simulink model "VoltageSourceConverterHVDCTrans"  (R2025b)
settings: Solver=FixedStepDiscrete  StartTime=0.0  StopTime=5  FixedStep=Ts  MaxStep=1e-4  RelTol=1e-3
PreLoadFcn:
  | VoltageSourceConverterHVDCTransParameters
values from neighbouring files (symbols this model uses):
  c = 0.207e-6    (= 2.07e-07)    [VoltageSourceConverterHVDCTransParameters.m]
  Cf = ((QRatedFilter/(VRated^2*(2*pi*FRated)))*(n^2-1)/(n^2))/Cbase    [VoltageSourceConverterHVDCTransParameters.m]
  FRated = 60    [VoltageSourceConverterHVDCTransParameters.m]
  Idcbase = Pbase/VdcRated    (= 1000)    [VoltageSourceConverterHVDCTransParameters.m]
  IL0 = opIdc.get("I").Value.value    [VoltageSourceConverterHVDCTransInitializeModel.m]
  l = 0.189e-3    (= 0.000189)    [VoltageSourceConverterHVDCTransParameters.m]
  Lbase = Zbase/wbase    [VoltageSourceConverterHVDCTransParameters.m]
  Lr = 0.15    [VoltageSourceConverterHVDCTransParameters.m]
  n = 25    [VoltageSourceConverterHVDCTransParameters.m]
  PRated = 300e6    (= 300000000)    [VoltageSourceConverterHVDCTransParameters.m]
  r = 0.0376    [VoltageSourceConverterHVDCTransParameters.m]
  Rc = r*Dis    (= 11.28)    [VoltageSourceConverterHVDCTransParameters.m]
  Rr = 0.002    [VoltageSourceConverterHVDCTransParameters.m]
  Rt = 0.002625    [VoltageSourceConverterHVDCTransParameters.m]
  Ts = 1/(fsw*100)    [VoltageSourceConverterHVDCTransInitializeModel.m]    (also in VoltageSourceConverterHVDCTransParameters.m = 6.66666666667e-05; VoltageSourceConverterHVDCTransVariantControl.m)
  Tsc = 10*Ts    (= 0.166666666667)    [VoltageSourceConverterHVDCTransInitializeModel.m]    (also in VoltageSourceConverterHVDCTransParameters.m = 6.66666666667e-05; VoltageSourceConverterHVDCTransVariantControl.m)
  Vdcr0 = 2*opReceivingEndVdcp.get("V").Value.value    [VoltageSourceConverterHVDCTransInitializeModel.m]
  VdcRated = 300e3    (= 300000)    [VoltageSourceConverterHVDCTransParameters.m]
  Vdcs0 = 2*opSendingEndVdcp.get("V").Value.value    [VoltageSourceConverterHVDCTransInitializeModel.m]
  VRated = 150e3    (= 150000)    [VoltageSourceConverterHVDCTransParameters.m]
  Xt = 0.19197    [VoltageSourceConverterHVDCTransParameters.m]
  Zbase = Vbase/Ibase    [VoltageSourceConverterHVDCTransParameters.m]
undefined symbols (not defined in the file or in its folder): DiscIntNeverNeededParam
libraries: nesl_utility x43, fl_lib x32, ee_lib x22, eeTransforms x16, eeGeneralControl x14, slpidlib x13, mcbeeMathTransformLib x8, eeSinusoidalMeasurement x2, eePwmGeneratorThreeLevel x2
(part 3 of 4)

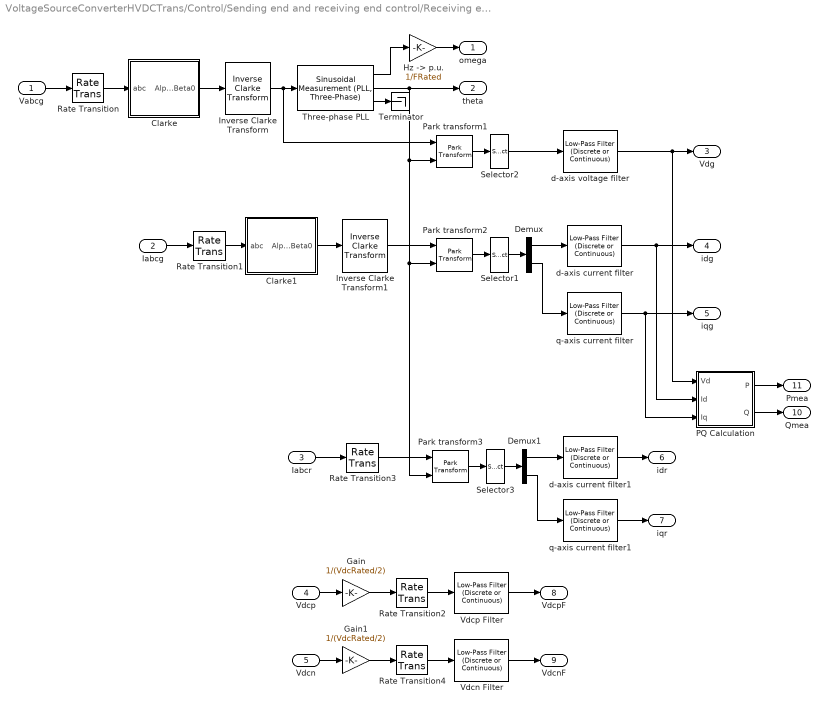
== system VoltageSourceConverterHVDCTrans/Control/Sending end and receiving end control/Receiving end control/Time mode/Measurements ==
  Vabcg : Inport
  Iabcg : Inport  Port=2
  Iabcr : Inport  Port=3
  Vdcp : Inport  Port=4
  Vdcn : Inport  Port=5
  Clarke : Subsystem
  Clarke1 : Subsystem
  Demux : Demux  Outputs=2
  Demux1 : Demux  Outputs=2
  Gain : Gain  Gain=1/(VdcRated/2)
  Gain1 : Gain  Gain=1/(VdcRated/2)
  "Hz -> p.u." : Gain  Gain=1/FRated
  Inverse Clarke Transform : mcbeeMathTransformLib/Inverse Clarke Transform  PowerInvariant=off  UseWithEmbedded=off  PhaseInput=Two inputs
      settings: LibrarySourceBlock=|
      | ee_sl_lib/Mathematical
      | Transforms/Inverse
      | Clarke Transform
  Inverse Clarke Transform1 : mcbeeMathTransformLib/Inverse Clarke Transform  PowerInvariant=off  UseWithEmbedded=off  PhaseInput=Two inputs
      settings: LibrarySourceBlock=|
      | ee_sl_lib/Mathematical
      | Transforms/Inverse
      | Clarke Transform
  PQ Calculation : Subsystem
  Park transform1 : eeTransforms/Park Transform  AxisAlignment=Q-axis  PowerInvariant=off
  Park transform2 : eeTransforms/Park Transform  AxisAlignment=Q-axis  PowerInvariant=off
  Park transform3 : eeTransforms/Park Transform  AxisAlignment=Q-axis  PowerInvariant=off
  Rate Transition : RateTransition  InitialCondition=Vabcgr0  OutPortSampleTime=Tsc
  Rate Transition1 : RateTransition  InitialCondition=Iabcgs0  OutPortSampleTime=Tsc
  Rate Transition2 : RateTransition  InitialCondition=Vdcr0/2/(VdcRated/2)  OutPortSampleTime=Tsc
  Rate Transition3 : RateTransition  InitialCondition=Iabcrs0  OutPortSampleTime=Tsc
  Rate Transition4 : RateTransition  InitialCondition=Vdcr0/2/(VdcRated/2)  OutPortSampleTime=Tsc
  Selector1 : Selector  InputPortWidth=3  IndexOptions=Index vector (dialog)  Indices=[1 2]  OutputSizes=1
  Selector2 : Selector  InputPortWidth=3  IndexOptions=Index vector (dialog)  Indices=[1]  OutputSizes=1
  Selector3 : Selector  InputPortWidth=3  IndexOptions=Index vector (dialog)  Indices=[1 2]  OutputSizes=1
  Terminator : Terminator
  Three-phase PLL : eeSinusoidalMeasurement/Sinusoidal Measurement (PLL, Three-Phase)  Kp_LF=45  Ki_LF=1250  F0=60  Theta0=-pi/6+Vphaser0  Ts=Tsc
  Vdcn Filter : eeGeneralControl/Low-Pass Filter (Discrete or Continuous)  K=1  T=5e-3  B=inf  A=-inf  init_option=Specify as parameter  x0=Vdcr0/2/(VdcRated/2)  Ts=Tsc
  Vdcp Filter : eeGeneralControl/Low-Pass Filter (Discrete or Continuous)  K=1  T=5e-3  B=inf  A=-inf  init_option=Specify as parameter  x0=Vdcr0/2/(VdcRated/2)  Ts=Tsc
  d-axis current filter : eeGeneralControl/Low-Pass Filter (Discrete or Continuous)  K=1  T=5e-3  B=inf  A=-inf  init_option=Specify as parameter  x0=Idgr0  Ts=Tsc
  d-axis current filter1 : eeGeneralControl/Low-Pass Filter (Discrete or Continuous)  K=1  T=5e-3  B=inf  A=-inf  init_option=Specify as parameter  x0=Idr0  Ts=Tsc
  d-axis voltage filter : eeGeneralControl/Low-Pass Filter (Discrete or Continuous)  K=1  T=5e-3  B=inf  A=-inf  init_option=Specify as parameter  x0=Vdgr0  Ts=Tsc
  q-axis current filter : eeGeneralControl/Low-Pass Filter (Discrete or Continuous)  K=1  T=5e-3  B=inf  A=-inf  init_option=Specify as parameter  x0=Iqgr0  Ts=Tsc
  q-axis current filter1 : eeGeneralControl/Low-Pass Filter (Discrete or Continuous)  K=1  T=5e-3  B=inf  A=-inf  init_option=Specify as parameter  x0=Iqr0  Ts=Tsc
  omega : Outport  VectorParamsAs1DForOutWhenUnconnected=off
  theta : Outport  Port=2  VectorParamsAs1DForOutWhenUnconnected=off
  Vdg : Outport  Port=3  VectorParamsAs1DForOutWhenUnconnected=off
  idg : Outport  Port=4  VectorParamsAs1DForOutWhenUnconnected=off
  iqg : Outport  Port=5  VectorParamsAs1DForOutWhenUnconnected=off
  idr : Outport  Port=6  VectorParamsAs1DForOutWhenUnconnected=off
  iqr : Outport  Port=7  VectorParamsAs1DForOutWhenUnconnected=off
  VdcpF : Outport  Port=8  VectorParamsAs1DForOutWhenUnconnected=off
  VdcnF : Outport  Port=9  VectorParamsAs1DForOutWhenUnconnected=off
  Qmea : Outport  Port=10  VectorParamsAs1DForOutWhenUnconnected=off
  Pmea : Outport  Port=11  VectorParamsAs1DForOutWhenUnconnected=off
  wires:
  Vdcn Filter/1 -> VdcnF/1
  Vdcn/1 -> Gain1/1
  Rate Transition4/1 -> Vdcn Filter/1
  Gain1/1 -> Rate Transition4/1
  q-axis current filter1/1 -> iqr/1
  d-axis current filter1/1 -> idr/1
  Demux1/2 -> q-axis current filter1/1
  Demux1/1 -> d-axis current filter1/1
  Rate Transition3/1 -> Park transform3/1
  Selector3/1 -> Demux1/1
  Park transform3/1 -> Selector3/1
  Iabcr/1 -> Rate Transition3/1
  PQ Calculation/2(Q) -> Qmea/1
  PQ Calculation/1(P) -> Pmea/1
  Selector2/1 -> d-axis voltage filter/1
  d-axis current filter/1 -> idg/1, PQ Calculation/2(Id)
  Inverse Clarke Transform1/1 -> Park transform2/1
  Clarke1/1(AlphaBeta0) -> Inverse Clarke Transform1/1
  Inverse Clarke Transform/1 -> Park transform1/1, Three-phase PLL/1
  Clarke/1(AlphaBeta0) -> Inverse Clarke Transform/1
  d-axis voltage filter/1 -> PQ Calculation/1(Vd), Vdg/1
  Park transform2/1 -> Selector1/1
  Demux/1 -> d-axis current filter/1
  Rate Transition/1 -> Clarke/1(abc)
  Gain/1 -> Rate Transition2/1
  Vdcp/1 -> Gain/1
  Demux/2 -> q-axis current filter/1
  Three-phase PLL/1 -> "Hz -> p.u."/1
  Park transform1/1 -> Selector2/1
  Three-phase PLL/2 -> Park transform1/2, Park transform3/2, Park transform2/2, theta/1
  Selector1/1 -> Demux/1
  Three-phase PLL/3 -> Terminator/1
  Vdcp Filter/1 -> VdcpF/1
  "Hz -> p.u."/1 -> omega/1
  Iabcg/1 -> Rate Transition1/1
  Vabcg/1 -> Rate Transition/1
  Rate Transition2/1 -> Vdcp Filter/1
  Rate Transition1/1 -> Clarke1/1(abc)
  q-axis current filter/1 -> iqg/1, PQ Calculation/3(Iq)

== system VoltageSourceConverterHVDCTrans/Control/Sending end and receiving end control/Receiving end control/Time mode/Receiving-end Control ==
  VdcRef : Inport
  Qref : Inport  Port=2
  omega : Inport  Port=3
  theta : Inport  Port=4
  Vd : Inport  Port=5
  idg : Inport  Port=6
  iqg : Inport  Port=7
  idr : Inport  Port=8
  iqr : Inport  Port=9
  Vdcp : Inport  Port=10
  Vdcn : Inport  Port=11
  Qmea : Inport  Port=12
  Current control : Subsystem
  DC voltage and reactive power control : Subsystem
  Unit Delay : UnitDelay  InitialCondition=Idgr0  SampleTime=Tsc  HasFrameUpgradeWarning=on
  Unit Delay1 : UnitDelay  InitialCondition=Iqgr0  SampleTime=Tsc  HasFrameUpgradeWarning=on
  Unit Delay2 : UnitDelay  InitialCondition=1  SampleTime=Tsc  HasFrameUpgradeWarning=on
  Unit Delay3 : UnitDelay  InitialCondition=Vdcr0/2/(VdcRated/2)  SampleTime=Tsc  HasFrameUpgradeWarning=on
  Unit Delay4 : UnitDelay  InitialCondition=Vdcr0/2/(VdcRated/2)  SampleTime=Tsc  HasFrameUpgradeWarning=on
  S : Outport
  wires:
  DC voltage and reactive power control/2(iqRef) -> Current control/2(iqgRef)
  DC voltage and reactive power control/1(idRef) -> Current control/1(idgRef)
  idg/1 -> Unit Delay/1
  iqg/1 -> Unit Delay1/1
  theta/1 -> Current control/11(theta)
  Vd/1 -> Current control/7(Vd)
  omega/1 -> Unit Delay2/1
  Current control/1(S) -> S/1
  Unit Delay/1 -> Current control/3(idg)
  Unit Delay1/1 -> Current control/4(iqg)
  Unit Delay2/1 -> Current control/10(omega)
  idr/1 -> Current control/5(idr)
  iqr/1 -> Current control/6(iqr)
  Vdcp/1 -> Unit Delay3/1
  VdcRef/1 -> DC voltage and reactive power control/1(VdcRef)
  Qref/1 -> DC voltage and reactive power control/4(Qref)
  Qmea/1 -> DC voltage and reactive power control/5(Qmea)
  Vdcn/1 -> Unit Delay4/1
  Unit Delay3/1 -> DC voltage and reactive power control/2(Vdcp), Current control/8(Vdcp)
  Unit Delay4/1 -> DC voltage and reactive power control/3(Vdcn), Current control/9(Vdcn)

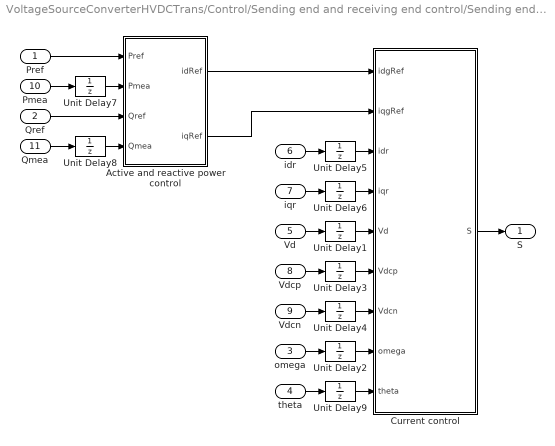
== system VoltageSourceConverterHVDCTrans/Control/Sending end and receiving end control/Sending end control/Frequency-and-time mode/Control ==
  Pref : Inport
  Qref : Inport  Port=2
  omega : Inport  Port=3
  theta : Inport  Port=4
  Vd : Inport  Port=5
  idr : Inport  Port=6
  iqr : Inport  Port=7
  Vdcp : Inport  Port=8
  Vdcn : Inport  Port=9
  Pmea : Inport  Port=10
  Qmea : Inport  Port=11
  Active and reactive power control : Subsystem
  Current control : Subsystem
  Unit Delay1 : UnitDelay  InitialCondition=Vdgs0  SampleTime=Tsc  HasFrameUpgradeWarning=on
  Unit Delay2 : UnitDelay  InitialCondition=1  SampleTime=Tsc  HasFrameUpgradeWarning=on
  Unit Delay3 : UnitDelay  InitialCondition=Vdcs0/2/(VdcRated/2)  SampleTime=Tsc  HasFrameUpgradeWarning=on
  Unit Delay4 : UnitDelay  InitialCondition=Vdcs0/2/(VdcRated/2)  SampleTime=Tsc  HasFrameUpgradeWarning=on
  Unit Delay5 : UnitDelay  InitialCondition=Ids0  SampleTime=Tsc  HasFrameUpgradeWarning=on
  Unit Delay6 : UnitDelay  InitialCondition=Iqs0  SampleTime=Tsc  HasFrameUpgradeWarning=on
  Unit Delay7 : UnitDelay  InitialCondition=Ps0  SampleTime=Tsc  HasFrameUpgradeWarning=on
  Unit Delay8 : UnitDelay  InitialCondition=Qs0  SampleTime=Tsc  HasFrameUpgradeWarning=on
  Unit Delay9 : UnitDelay  InitialCondition=-pi/6+Vphases0  SampleTime=Tsc  HasFrameUpgradeWarning=on
  S : Outport
  wires:
  Current control/1(S) -> S/1
  Unit Delay5/1 -> Current control/3(idr)
  Unit Delay3/1 -> Current control/6(Vdcp)
  Unit Delay2/1 -> Current control/8(omega)
  Unit Delay6/1 -> Current control/4(iqr)
  Unit Delay8/1 -> Active and reactive power control/4(Qmea)
  Unit Delay7/1 -> Active and reactive power control/2(Pmea)
  Active and reactive power control/2(iqRef) -> Current control/2(iqgRef)
  Unit Delay1/1 -> Current control/5(Vd)
  Active and reactive power control/1(idRef) -> Current control/1(idgRef)
  iqr/1 -> Unit Delay6/1
  Vd/1 -> Unit Delay1/1
  Unit Delay4/1 -> Current control/7(Vdcn)
  Qmea/1 -> Unit Delay8/1
  Vdcp/1 -> Unit Delay3/1
  Vdcn/1 -> Unit Delay4/1
  idr/1 -> Unit Delay5/1
  theta/1 -> Unit Delay9/1
  omega/1 -> Unit Delay2/1
  Qref/1 -> Active and reactive power control/3(Qref)
  Pref/1 -> Active and reactive power control/1(Pref)
  Pmea/1 -> Unit Delay7/1
  Unit Delay9/1 -> Current control/9(theta)

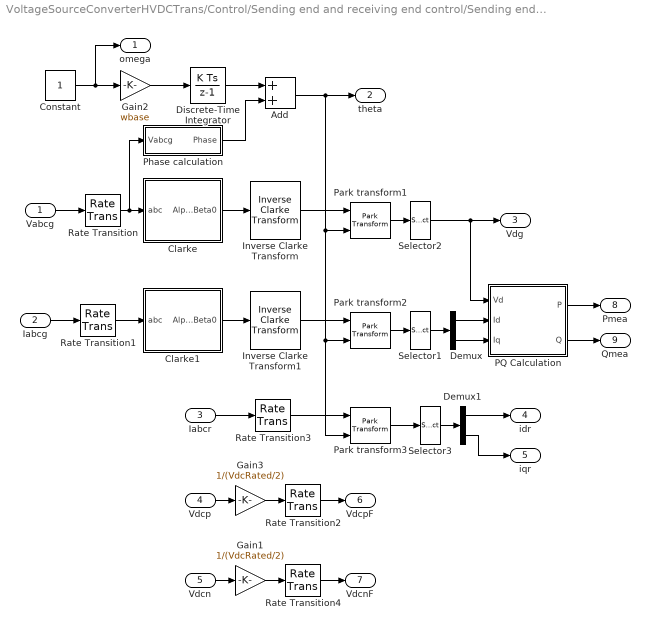
== system VoltageSourceConverterHVDCTrans/Control/Sending end and receiving end control/Sending end control/Frequency-and-time mode/Measurements ==
  Vabcg : Inport
  Iabcg : Inport  Port=2
  Iabcr : Inport  Port=3
  Vdcp : Inport  Port=4
  Vdcn : Inport  Port=5
  Add : Sum
  Clarke : Subsystem
  Clarke1 : Subsystem
  Constant : Constant  SampleTime=Tsc
  Demux : Demux  Outputs=2
  Demux1 : Demux  Outputs=2
  Discrete-Time Integrator : DiscreteIntegrator  InitialCondition=-pi/6  SampleTime=Tsc  ICPrevOutput=DiscIntNeverNeededParam  ICPrevScaledInput=DiscIntNeverNeededParam
  Gain1 : Gain  Gain=1/(VdcRated/2)
  Gain2 : Gain  Gain=wbase
  Gain3 : Gain  Gain=1/(VdcRated/2)
  Inverse Clarke Transform : mcbeeMathTransformLib/Inverse Clarke Transform  PowerInvariant=off  UseWithEmbedded=off  PhaseInput=Two inputs
      settings: LibrarySourceBlock=|
      | ee_sl_lib/Mathematical
      | Transforms/Inverse
      | Clarke Transform
  Inverse Clarke Transform1 : mcbeeMathTransformLib/Inverse Clarke Transform  PowerInvariant=off  UseWithEmbedded=off  PhaseInput=Two inputs
      settings: LibrarySourceBlock=|
      | ee_sl_lib/Mathematical
      | Transforms/Inverse
      | Clarke Transform
  PQ Calculation : Subsystem
  Park transform1 : eeTransforms/Park Transform  AxisAlignment=Q-axis  PowerInvariant=off
  Park transform2 : eeTransforms/Park Transform  AxisAlignment=Q-axis  PowerInvariant=off
  Park transform3 : eeTransforms/Park Transform  AxisAlignment=Q-axis  PowerInvariant=off
  Phase calculation : Subsystem
  Rate Transition : RateTransition  InitialCondition=Vabcgs0  OutPortSampleTime=Tsc
  Rate Transition1 : RateTransition  InitialCondition=Iabcgs0  OutPortSampleTime=Tsc
  Rate Transition2 : RateTransition  InitialCondition=Vdcs0/2/(VdcRated/2)  OutPortSampleTime=Tsc
  Rate Transition3 : RateTransition  InitialCondition=Iabcrs0  OutPortSampleTime=Tsc
  Rate Transition4 : RateTransition  InitialCondition=Vdcs0/2/(VdcRated/2)  OutPortSampleTime=Tsc
  Selector1 : Selector  InputPortWidth=3  IndexOptions=Index vector (dialog)  Indices=[1 2]  OutputSizes=1
  Selector2 : Selector  InputPortWidth=3  IndexOptions=Index vector (dialog)  Indices=[1]  OutputSizes=1
  Selector3 : Selector  InputPortWidth=3  IndexOptions=Index vector (dialog)  Indices=[1 2]  OutputSizes=1
  omega : Outport  VectorParamsAs1DForOutWhenUnconnected=off
  theta : Outport  Port=2  VectorParamsAs1DForOutWhenUnconnected=off
  Vdg : Outport  Port=3  VectorParamsAs1DForOutWhenUnconnected=off
  idr : Outport  Port=4  VectorParamsAs1DForOutWhenUnconnected=off
  iqr : Outport  Port=5  VectorParamsAs1DForOutWhenUnconnected=off
  VdcpF : Outport  Port=6  VectorParamsAs1DForOutWhenUnconnected=off
  VdcnF : Outport  Port=7  VectorParamsAs1DForOutWhenUnconnected=off
  Pmea : Outport  Port=8  VectorParamsAs1DForOutWhenUnconnected=off
  Qmea : Outport  Port=9  VectorParamsAs1DForOutWhenUnconnected=off
  wires:
  Park transform3/1 -> Selector3/1
  Selector3/1 -> Demux1/1
  Rate Transition1/1 -> Clarke1/1(abc)
  PQ Calculation/1(P) -> Pmea/1
  Clarke/1(AlphaBeta0) -> Inverse Clarke Transform/1
  Selector1/1 -> Demux/1
  Vdcp/1 -> Gain3/1
  Add/1 -> theta/1, Park transform3/2, Park transform2/2, Park transform1/2
  PQ Calculation/2(Q) -> Qmea/1
  Demux/2 -> PQ Calculation/3(Iq)
  Vabcg/1 -> Rate Transition/1
  Rate Transition4/1 -> VdcnF/1
  Iabcr/1 -> Rate Transition3/1
  Inverse Clarke Transform/1 -> Park transform1/1
  Vdcn/1 -> Gain1/1
  Park transform2/1 -> Selector1/1
  Rate Transition/1 -> Phase calculation/1(Vabcg), Clarke/1(abc)
  Demux1/1 -> idr/1
  Demux1/2 -> iqr/1
  Park transform1/1 -> Selector2/1
  Gain1/1 -> Rate Transition4/1
  Rate Transition2/1 -> VdcpF/1
  Iabcg/1 -> Rate Transition1/1
  Clarke1/1(AlphaBeta0) -> Inverse Clarke Transform1/1
  Constant/1 -> omega/1, Gain2/1
  Selector2/1 -> Vdg/1, PQ Calculation/1(Vd)
  Inverse Clarke Transform1/1 -> Park transform2/1
  Gain3/1 -> Rate Transition2/1
  Demux/1 -> PQ Calculation/2(Id)
  Gain2/1 -> Discrete-Time Integrator/1
  Rate Transition3/1 -> Park transform3/1
  Discrete-Time Integrator/1 -> Add/1
  Phase calculation/1(Phase) -> Add/2

== system VoltageSourceConverterHVDCTrans/Control/Sending end and receiving end control/Sending end control/Time mode/Control ==
  Pref : Inport
  Qref : Inport  Port=2
  omega : Inport  Port=3
  theta : Inport  Port=4
  Vd : Inport  Port=5
  idg : Inport  Port=6
  iqg : Inport  Port=7
  idr : Inport  Port=8
  iqr : Inport  Port=9
  Vdcp : Inport  Port=10
  Vdcn : Inport  Port=11
  Pmea : Inport  Port=12
  Qmea : Inport  Port=13
  Active and reactive power control : Subsystem
  Current control : Subsystem
  Unit Delay : UnitDelay  InitialCondition=Idgs0  SampleTime=Tsc  HasFrameUpgradeWarning=on
  Unit Delay1 : UnitDelay  InitialCondition=Iqgs0  SampleTime=Tsc  HasFrameUpgradeWarning=on
  Unit Delay2 : UnitDelay  InitialCondition=1  SampleTime=Tsc  HasFrameUpgradeWarning=on
  Unit Delay3 : UnitDelay  InitialCondition=Vdcs0/2/(VdcRated/2)  SampleTime=Tsc  HasFrameUpgradeWarning=on
  Unit Delay4 : UnitDelay  InitialCondition=Vdcs0/2/(VdcRated/2)  SampleTime=Tsc  HasFrameUpgradeWarning=on
  S : Outport
  wires:
  idg/1 -> Unit Delay/1
  iqg/1 -> Unit Delay1/1
  theta/1 -> Current control/11(theta)
  Vd/1 -> Current control/7(Vd)
  omega/1 -> Unit Delay2/1
  Current control/1(S) -> S/1
  Unit Delay/1 -> Current control/3(idg)
  Unit Delay1/1 -> Current control/4(iqg)
  Unit Delay2/1 -> Current control/10(omega)
  idr/1 -> Current control/5(idr)
  iqr/1 -> Current control/6(iqr)
  Vdcp/1 -> Unit Delay3/1
  Pref/1 -> Active and reactive power control/1(Pref)
  Pmea/1 -> Active and reactive power control/2(Pmea)
  Qref/1 -> Active and reactive power control/3(Qref)
  Qmea/1 -> Active and reactive power control/4(Qmea)
  Active and reactive power control/1(idRef) -> Current control/1(idgRef)
  Active and reactive power control/2(iqRef) -> Current control/2(iqgRef)
  Vdcn/1 -> Unit Delay4/1
  Unit Delay3/1 -> Current control/8(Vdcp)
  Unit Delay4/1 -> Current control/9(Vdcn)

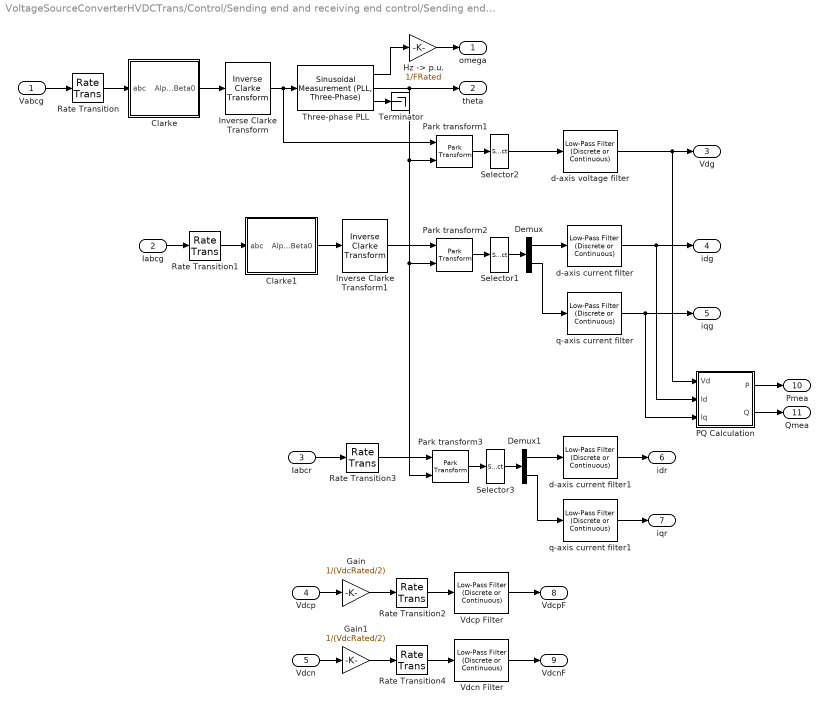
== system VoltageSourceConverterHVDCTrans/Control/Sending end and receiving end control/Sending end control/Time mode/Measurements ==
  Vabcg : Inport
  Iabcg : Inport  Port=2
  Iabcr : Inport  Port=3
  Vdcp : Inport  Port=4
  Vdcn : Inport  Port=5
  Clarke : Subsystem
  Clarke1 : Subsystem
  Demux : Demux  Outputs=2
  Demux1 : Demux  Outputs=2
  Gain : Gain  Gain=1/(VdcRated/2)
  Gain1 : Gain  Gain=1/(VdcRated/2)
  "Hz -> p.u." : Gain  Gain=1/FRated
  Inverse Clarke Transform : mcbeeMathTransformLib/Inverse Clarke Transform  PowerInvariant=off  UseWithEmbedded=off  PhaseInput=Two inputs
      settings: LibrarySourceBlock=|
      | ee_sl_lib/Mathematical
      | Transforms/Inverse
      | Clarke Transform
  Inverse Clarke Transform1 : mcbeeMathTransformLib/Inverse Clarke Transform  PowerInvariant=off  UseWithEmbedded=off  PhaseInput=Two inputs
      settings: LibrarySourceBlock=|
      | ee_sl_lib/Mathematical
      | Transforms/Inverse
      | Clarke Transform
  PQ Calculation : Subsystem
  Park transform1 : eeTransforms/Park Transform  AxisAlignment=Q-axis  PowerInvariant=off
  Park transform2 : eeTransforms/Park Transform  AxisAlignment=Q-axis  PowerInvariant=off
  Park transform3 : eeTransforms/Park Transform  AxisAlignment=Q-axis  PowerInvariant=off
  Rate Transition : RateTransition  InitialCondition=Vabcgs0  OutPortSampleTime=Tsc
  Rate Transition1 : RateTransition  InitialCondition=Iabcgs0  OutPortSampleTime=Tsc
  Rate Transition2 : RateTransition  InitialCondition=Vdcs0/2/(VdcRated/2)  OutPortSampleTime=Tsc
  Rate Transition3 : RateTransition  InitialCondition=Iabcrs0  OutPortSampleTime=Tsc
  Rate Transition4 : RateTransition  InitialCondition=Vdcs0/2/(VdcRated/2)  OutPortSampleTime=Tsc
  Selector1 : Selector  InputPortWidth=3  IndexOptions=Index vector (dialog)  Indices=[1 2]  OutputSizes=1
  Selector2 : Selector  InputPortWidth=3  IndexOptions=Index vector (dialog)  Indices=[1]  OutputSizes=1
  Selector3 : Selector  InputPortWidth=3  IndexOptions=Index vector (dialog)  Indices=[1 2]  OutputSizes=1
  Terminator : Terminator
  Three-phase PLL : eeSinusoidalMeasurement/Sinusoidal Measurement (PLL, Three-Phase)  Kp_LF=45  Ki_LF=1250  F0=60  Theta0=-pi/6+Vphases0  Ts=Tsc
  Vdcn Filter : eeGeneralControl/Low-Pass Filter (Discrete or Continuous)  K=1  T=5e-3  B=inf  A=-inf  init_option=Specify as parameter  x0=Vdcs0/2/(VdcRated/2)  Ts=Tsc
  Vdcp Filter : eeGeneralControl/Low-Pass Filter (Discrete or Continuous)  K=1  T=5e-3  B=inf  A=-inf  init_option=Specify as parameter  x0=Vdcs0/2/(VdcRated/2)  Ts=Tsc
  d-axis current filter : eeGeneralControl/Low-Pass Filter (Discrete or Continuous)  K=1  T=5e-3  B=inf  A=-inf  init_option=Specify as parameter  x0=Idgs0  Ts=Tsc
  d-axis current filter1 : eeGeneralControl/Low-Pass Filter (Discrete or Continuous)  K=1  T=5e-3  B=inf  A=-inf  init_option=Specify as parameter  x0=Ids0  Ts=Tsc
  d-axis voltage filter : eeGeneralControl/Low-Pass Filter (Discrete or Continuous)  K=1  T=5e-3  B=inf  A=-inf  init_option=Specify as parameter  x0=Vdgs0  Ts=Tsc
  q-axis current filter : eeGeneralControl/Low-Pass Filter (Discrete or Continuous)  K=1  T=5e-3  B=inf  A=-inf  init_option=Specify as parameter  x0=Iqgs0  Ts=Tsc
  q-axis current filter1 : eeGeneralControl/Low-Pass Filter (Discrete or Continuous)  K=1  T=5e-3  B=inf  A=-inf  init_option=Specify as parameter  x0=Iqs0  Ts=Tsc
  omega : Outport  VectorParamsAs1DForOutWhenUnconnected=off
  theta : Outport  Port=2  VectorParamsAs1DForOutWhenUnconnected=off
  Vdg : Outport  Port=3  VectorParamsAs1DForOutWhenUnconnected=off
  idg : Outport  Port=4  VectorParamsAs1DForOutWhenUnconnected=off
  iqg : Outport  Port=5  VectorParamsAs1DForOutWhenUnconnected=off
  idr : Outport  Port=6  VectorParamsAs1DForOutWhenUnconnected=off
  iqr : Outport  Port=7  VectorParamsAs1DForOutWhenUnconnected=off
  VdcpF : Outport  Port=8  VectorParamsAs1DForOutWhenUnconnected=off
  VdcnF : Outport  Port=9  VectorParamsAs1DForOutWhenUnconnected=off
  Pmea : Outport  Port=10  VectorParamsAs1DForOutWhenUnconnected=off
  Qmea : Outport  Port=11  VectorParamsAs1DForOutWhenUnconnected=off
  wires:
  q-axis current filter/1 -> PQ Calculation/3(Iq), iqg/1
  Rate Transition1/1 -> Clarke1/1(abc)
  Rate Transition2/1 -> Vdcp Filter/1
  Vabcg/1 -> Rate Transition/1
  Iabcg/1 -> Rate Transition1/1
  "Hz -> p.u."/1 -> omega/1
  Vdcp Filter/1 -> VdcpF/1
  Three-phase PLL/3 -> Terminator/1
  Selector1/1 -> Demux/1
  Three-phase PLL/2 -> theta/1, Park transform2/2, Park transform3/2, Park transform1/2
  Park transform1/1 -> Selector2/1
  Three-phase PLL/1 -> "Hz -> p.u."/1
  Demux/2 -> q-axis current filter/1
  Vdcp/1 -> Gain/1
  Gain/1 -> Rate Transition2/1
  Rate Transition/1 -> Clarke/1(abc)
  Demux/1 -> d-axis current filter/1
  Park transform2/1 -> Selector1/1
  d-axis voltage filter/1 -> Vdg/1, PQ Calculation/1(Vd)
  Clarke/1(AlphaBeta0) -> Inverse Clarke Transform/1
  Inverse Clarke Transform/1 -> Three-phase PLL/1, Park transform1/1
  Clarke1/1(AlphaBeta0) -> Inverse Clarke Transform1/1
  Inverse Clarke Transform1/1 -> Park transform2/1
  d-axis current filter/1 -> PQ Calculation/2(Id), idg/1
  Selector2/1 -> d-axis voltage filter/1
  PQ Calculation/1(P) -> Pmea/1
  PQ Calculation/2(Q) -> Qmea/1
  Iabcr/1 -> Rate Transition3/1
  Park transform3/1 -> Selector3/1
  Selector3/1 -> Demux1/1
  Rate Transition3/1 -> Park transform3/1
  Demux1/1 -> d-axis current filter1/1
  Demux1/2 -> q-axis current filter1/1
  d-axis current filter1/1 -> idr/1
  q-axis current filter1/1 -> iqr/1
  Gain1/1 -> Rate Transition4/1
  Rate Transition4/1 -> Vdcn Filter/1
  Vdcn/1 -> Gain1/1
  Vdcn Filter/1 -> VdcnF/1

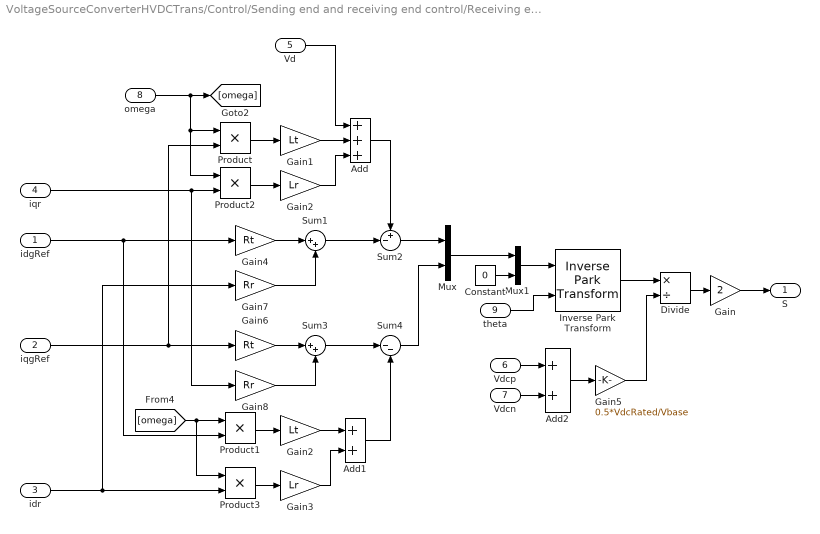
== system VoltageSourceConverterHVDCTrans/Control/Sending end and receiving end control/Receiving end control/Frequency-and-time mode/Control/Current control ==
  idgRef : Inport
  iqgRef : Inport  Port=2
  idr : Inport  Port=3
  iqr : Inport  Port=4
  Vd : Inport  Port=5
  Vdcp : Inport  Port=6
  Vdcn : Inport  Port=7
  omega : Inport  Port=8
  theta : Inport  Port=9
  Add : Sum  Inputs=+++
  Add1 : Sum
  Add2 : Sum
  Constant : Constant  Value=0  SampleTime=Tsc
  Divide : Product  Inputs=*/
  Gain : Gain  Gain=2
  Gain1 : Gain  Gain=Lt
  Gain2 : Gain  Gain=Lr
  "Gain2 " : Gain  Gain=Lt
  Gain3 : Gain  Gain=Lr
  Gain4 : Gain  Gain=Rt
  Gain5 : Gain  Gain=0.5*VdcRated/Vbase
  Gain6 : Gain  Gain=Rt
  Gain7 : Gain  Gain=Rr
  Gain8 : Gain  Gain=Rr
  Inverse Park Transform : eeTransforms/Inverse Park Transform  AxisAlignment=Q-axis  PowerInvariant=off
  Mux : Mux  Inputs=2
  Mux1 : Mux  Inputs=2
  Product{,1..3} (4 alike) : Product  Inputs=**
  Sum1 : Sum  Inputs=|++
  Sum2 : Sum  Inputs=+-|
  Sum3 : Sum  Inputs=|++
  Sum4 : Sum  Inputs=|--
  S : Outport
  wires:
  Vdcn/1 -> Add2/2
  Vdcp/1 -> Add2/1
  Gain8/1 -> Sum3/2
  Gain6/1 -> Sum3/1
  Gain7/1 -> Sum1/2
  Gain4/1 -> Sum1/1
  Gain/1 -> S/1
  Gain5/1 -> Divide/2
  Add2/1 -> Gain5/1
  Sum3/1 -> Sum4/1
  Sum1/1 -> Sum2/2
  Divide/1 -> Gain/1
  Add1/1 -> Sum4/2
  Gain3/1 -> Add1/2
  "Gain2 "/1 -> Add1/1
  Product3/1 -> Gain3/1
  idr/1 -> Product3/2, Gain7/1
  Gain2/1 -> Add/3
  Product2/1 -> Gain2/1
  iqr/1 -> Gain8/1, Product2/2
  Sum2/1 -> Mux/1
  Gain1/1 -> Add/2
  theta/1 -> Inverse Park Transform/2
  Add/1 -> Sum2/1
  Product1/1 -> "Gain2 "/1
  Sum4/1 -> Mux/2
  Product/1 -> Gain1/1
  [omega] -> Product1/1, Product3/1
  omega/1 -> [omega], Product/1, Product2/1
  iqgRef/1 -> Gain6/1, Product/2
  Mux1/1 -> Inverse Park Transform/1
  Inverse Park Transform/1 -> Divide/1
  Constant/1 -> Mux1/2
  idgRef/1 -> Gain4/1, Product1/2
  Mux/1 -> Mux1/1
  Vd/1 -> Add/1

== system VoltageSourceConverterHVDCTrans/Control/Sending end and receiving end control/Receiving end control/Frequency-and-time mode/Control/DC voltage and reactive power control ==
  VdcRef : Inport
  Vdcp : Inport  Port=2
  Vdcn : Inport  Port=3
  Qref : Inport  Port=4
  Qmea : Inport  Port=5
  Add2 : Sum
  Gain : Gain  Gain=-1
  Gain1 : Gain  Gain=VdcRated/Vbase
  Gain2 : Gain  Gain=0.5
  P PI : slpidlib/PID Controller  Controller=PI  Form=Parallel  TimeDomain=Discrete-time  UseExternalTs=off  SampleTime=Tsc  IntegratorMethod=Forward Euler  FilterMethod=Forward Euler  ControllerParametersSource=internal  P=REnd_Vdc_PI_Low(1)  I=REnd_Vdc_PI_Low(2)  UseKiTs=off  D=0  UseExternalDerivativeSource=off  N=100  UseFilter=on  TunerSelectOption=Transfer Function Based (PID Tuner App)  InitialConditionSource=internal  InitialConditionForIntegrator=P_PIr0  InitialConditionForFilter=0  DifferentiatorICPrevScaledInput=0  ExternalReset=none  TrackingMode=off  Kt=1  LimitOutput=on  SatLimitsSource=internal  UpperSaturationLimit=1.5  LowerSaturationLimit=-1.5  LinearizeAsGain=on  AntiWindupMode=back-calculation  Kb=1000  LimitIntegrator=off  UpperIntegratorSaturationLimit=inf  LowerIntegratorSaturationLimit=-inf  POutMin=[]  POutMax=[]  IOutMin=[]  IOutMax=[]  DOutMin=[]  DOutMax=[]  NOutMin=[]  NOutMax=[]  SumOutMin=[]  SumOutMax=[]  SaturationOutMin=[]  SaturationOutMax=[]  PParamMin=[]  PParamMax=[]  IParamMin=[]  IParamMax=[]  DParamMin=[]  DParamMax=[]  NParamMin=[]  NParamMax=[]  KbParamMin=[]  KbParamMax=[]  KtParamMin=[]  KtParamMax=[]  KbOutMin=[]  KbOutMax=[]  KtOutMin=[]  KtOutMax=[]  IntegratorOutMin=[]  IntegratorOutMax=[]  FilterOutMin=[]  FilterOutMax=[]  SumI1OutMin=[]  SumI1OutMax=[]  SumI2OutMin=[]  SumI2OutMax=[]  SumI3OutMin=[]  SumI3OutMax=[]  SumI4OutMin=[]  SumI4OutMax=[]  SumDOutMin=[]  SumDOutMax=[]  DifferentiatorOutMin=[]  DifferentiatorOutMax=[]  FilterDiffOutCoefMin=[]  FilterDiffOutCoefMax=[]  ReciprocalOutMin=[]  ReciprocalOutMax=[]  SumDenOutMin=[]  SumDenOutMax=[]  SumNumOutMin=[]  SumNumOutMax=[]  DivideOutMin=[]  DivideOutMax=[]  UdiffTsProdOutMin=[]  UdiffTsProdOutMax=[]  NTsProdOutMin=[]  NTsProdOutMax=[]  UintegralTsProdOutMin=[]  UintegralTsProdOutMax=[]  UngainTsProdOutMin=[]  UngainTsProdOutMax=[]  ClampingZeroOutDataTypeStr=Inherit: Inherit via back propagation  ClampingZeroOutMin=[]  ClampingZeroOutMax=[]  FilterDenConstantOutDataTypeStr=Inherit: Inherit via back propagation  FilterDenConstantOutMin=[]  FilterDenConstantOutMax=[]  PCopyOutDataTypeStr=Inherit: Inherit via back propagation  PCopyOutMin=[]  PCopyOutMax=[]  NCopyOutDataTypeStr=Inherit: Inherit via back propagation  NCopyOutMin=[]  NCopyOutMax=[]  IntegratorContinuousStateAttributes=''  IntegratorStateMustResolveToSignalObject=off  IntegratorRTWStateStorageClass=Auto  FilterContinuousStateAttributes=''  FilterStateMustResolveToSignalObject=off  FilterRTWStateStorageClass=Auto  ParallelPVariant=InternalParameters  IdealPVariant=Disabled  IVariant=InternalParameters  DVariant=Disabled  IntegratorVariant=Discrete  SatVariant=Enabled  AWVariant=BackCalculation  PCopyVariant=Disabled  TRVariant=Disabled  FdbkBlocksVariant=Forward  IdealPFdbkVariant=Disabled  SatFdbkVariant=Disabled  DerivativeFilterVariant=Disabled  NVariant=Disabled  NCopyVariant=Disabled_SignalSpec  FilterICVariant=Disabled  IntegratorICVariant=InternalICs  ExternalResetVariant=Disabled  TRSumVariant=Passthrough  SumFdbkVariant=Disabled  SumVariant=Sum_PI  TsampFilterVariant=InternalTs  TsampNgainVariant=Passthrough  TsampIntegralVariant=Disabled_SignalSpec  ExternalSaturationOutDataTypeStr=Inherit: Same as second input  DerivativeSourceVariant=Disabled  PreIntVariant=InternalPreInt
  Q PI : slpidlib/PID Controller  Controller=PI  Form=Parallel  TimeDomain=Discrete-time  UseExternalTs=off  SampleTime=Tsc  IntegratorMethod=Forward Euler  FilterMethod=Forward Euler  ControllerParametersSource=internal  P=REnd_Q_PI_Low(1)  I=REnd_Q_PI_Low(2)  UseKiTs=off  D=0  UseExternalDerivativeSource=off  N=100  UseFilter=on  TunerSelectOption=Transfer Function Based (PID Tuner App)  InitialConditionSource=internal  InitialConditionForIntegrator=-Q_PIr0  InitialConditionForFilter=0  DifferentiatorICPrevScaledInput=0  ExternalReset=none  TrackingMode=off  Kt=1  LimitOutput=on  SatLimitsSource=internal  UpperSaturationLimit=1.5  LowerSaturationLimit=-1.5  LinearizeAsGain=on  AntiWindupMode=back-calculation  Kb=1000  LimitIntegrator=off  UpperIntegratorSaturationLimit=inf  LowerIntegratorSaturationLimit=-inf  POutMin=[]  POutMax=[]  IOutMin=[]  IOutMax=[]  DOutMin=[]  DOutMax=[]  NOutMin=[]  NOutMax=[]  SumOutMin=[]  SumOutMax=[]  SaturationOutMin=[]  SaturationOutMax=[]  PParamMin=[]  PParamMax=[]  IParamMin=[]  IParamMax=[]  DParamMin=[]  DParamMax=[]  NParamMin=[]  NParamMax=[]  KbParamMin=[]  KbParamMax=[]  KtParamMin=[]  KtParamMax=[]  KbOutMin=[]  KbOutMax=[]  KtOutMin=[]  KtOutMax=[]  IntegratorOutMin=[]  IntegratorOutMax=[]  FilterOutMin=[]  FilterOutMax=[]  SumI1OutMin=[]  SumI1OutMax=[]  SumI2OutMin=[]  SumI2OutMax=[]  SumI3OutMin=[]  SumI3OutMax=[]  SumI4OutMin=[]  SumI4OutMax=[]  SumDOutMin=[]  SumDOutMax=[]  DifferentiatorOutMin=[]  DifferentiatorOutMax=[]  FilterDiffOutCoefMin=[]  FilterDiffOutCoefMax=[]  ReciprocalOutMin=[]  ReciprocalOutMax=[]  SumDenOutMin=[]  SumDenOutMax=[]  SumNumOutMin=[]  SumNumOutMax=[]  DivideOutMin=[]  DivideOutMax=[]  UdiffTsProdOutMin=[]  UdiffTsProdOutMax=[]  NTsProdOutMin=[]  NTsProdOutMax=[]  UintegralTsProdOutMin=[]  UintegralTsProdOutMax=[]  UngainTsProdOutMin=[]  UngainTsProdOutMax=[]  ClampingZeroOutDataTypeStr=Inherit: Inherit via back propagation  ClampingZeroOutMin=[]  ClampingZeroOutMax=[]  FilterDenConstantOutDataTypeStr=Inherit: Inherit via back propagation  FilterDenConstantOutMin=[]  FilterDenConstantOutMax=[]  PCopyOutDataTypeStr=Inherit: Inherit via back propagation  PCopyOutMin=[]  PCopyOutMax=[]  NCopyOutDataTypeStr=Inherit: Inherit via back propagation  NCopyOutMin=[]  NCopyOutMax=[]  IntegratorContinuousStateAttributes=''  IntegratorStateMustResolveToSignalObject=off  IntegratorRTWStateStorageClass=Auto  FilterContinuousStateAttributes=''  FilterStateMustResolveToSignalObject=off  FilterRTWStateStorageClass=Auto  ParallelPVariant=InternalParameters  IdealPVariant=Disabled  IVariant=InternalParameters  DVariant=Disabled  IntegratorVariant=Discrete  SatVariant=Enabled  AWVariant=BackCalculation  PCopyVariant=Disabled  TRVariant=Disabled  FdbkBlocksVariant=Forward  IdealPFdbkVariant=Disabled  SatFdbkVariant=Disabled  DerivativeFilterVariant=Disabled  NVariant=Disabled  NCopyVariant=Disabled_SignalSpec  FilterICVariant=Disabled  IntegratorICVariant=InternalICs  ExternalResetVariant=Disabled  TRSumVariant=Passthrough  SumFdbkVariant=Disabled  SumVariant=Sum_PI  TsampFilterVariant=InternalTs  TsampNgainVariant=Passthrough  TsampIntegralVariant=Disabled_SignalSpec  ExternalSaturationOutDataTypeStr=Inherit: Same as second input  DerivativeSourceVariant=Disabled  PreIntVariant=InternalPreInt
  Sum5 : Sum  Inputs=|+-
  Sum6 : Sum  Inputs=|+-
  idRef : Outport
  iqRef : Outport  Port=2
  wires:
  Sum5/1 -> Gain1/1
  P PI/1 -> idRef/1
  Sum6/1 -> Q PI/1
  Q PI/1 -> Gain/1
  Qref/1 -> Sum6/1
  Qmea/1 -> Sum6/2
  VdcRef/1 -> Sum5/1
  Gain/1 -> iqRef/1
  Add2/1 -> Gain2/1
  Vdcp/1 -> Add2/1
  Vdcn/1 -> Add2/2
  Gain2/1 -> Sum5/2
  Gain1/1 -> P PI/1

== system VoltageSourceConverterHVDCTrans/Control/Sending end and receiving end control/Receiving end control/Frequency-and-time mode/Measurements/Clarke ==
  abc : Inport
  0 : Fcn  Expr=u(1) + u(2) + u(3)
  K : Gain  Gain=[2 2 1]/3
  Mux : Mux  Inputs=3
  alpha : Fcn  Expr=(u(1) - u(3))*sqrt(3)/2
  beta : Fcn  Expr=-0.5*u(1) + u(2) -0.5*u(3)
  AlphaBeta0 : Outport
  wires:
  K/1 -> AlphaBeta0/1
  0/1 -> Mux/3
  alpha/1 -> Mux/1
  abc/1 -> 0/1, beta/1, alpha/1
  Mux/1 -> K/1
  beta/1 -> Mux/2

== system VoltageSourceConverterHVDCTrans/Control/Sending end and receiving end control/Receiving end control/Frequency-and-time mode/Measurements/Clarke1 ==
  abc : Inport
  0 : Fcn  Expr=u(1) + u(2) + u(3)
  K : Gain  Gain=[2 2 1]/3
  Mux : Mux  Inputs=3
  alpha : Fcn  Expr=(u(1) - u(3))*sqrt(3)/2
  beta : Fcn  Expr=-0.5*u(1) + u(2) -0.5*u(3)
  AlphaBeta0 : Outport
  wires:
  beta/1 -> Mux/2
  Mux/1 -> K/1
  abc/1 -> alpha/1, beta/1, 0/1
  alpha/1 -> Mux/1
  0/1 -> Mux/3
  K/1 -> AlphaBeta0/1

== system VoltageSourceConverterHVDCTrans/Control/Sending end and receiving end control/Receiving end control/Frequency-and-time mode/Measurements/PQ Calculation ==
  Vd : Inport
  Id : Inport  Port=2
  Iq : Inport  Port=3
  Gain : Gain  Gain=-1
  Product : Product
  Product4 : Product
  P : Outport
  Q : Outport  Port=2
  wires:
  Gain/1 -> Q/1
  Product4/1 -> Gain/1
  Iq/1 -> Product4/2
  Id/1 -> Product/2
  Product/1 -> P/1
  Vd/1 -> Product/1, Product4/1

== system VoltageSourceConverterHVDCTrans/Control/Sending end and receiving end control/Receiving end control/Frequency-and-time mode/Measurements/Phase calculation ==
  Vabcg : Inport
  Divide : Product  Inputs=*/
  Gain : Gain  Gain=2/3
  Math Function : Math  Operator=square
  Selector : Selector  InputPortWidth=3  IndexOptions=Index vector (dialog)  Indices=[1]  OutputSizes=1
  Sqrt : Sqrt
  Sum of Elements : Sum  Inputs=+
  Trigonometric Function : Trigonometry  Operator=asin
  Phase : Outport
  wires:
  Trigonometric Function/1 -> Phase/1
  Math Function/1 -> Sum of Elements/1
  Sum of Elements/1 -> Gain/1
  Selector/1 -> Divide/1
  Gain/1 -> Sqrt/1
  Vabcg/1 -> Math Function/1, Selector/1
  Divide/1 -> Trigonometric Function/1
  Sqrt/1 -> Divide/2

== system VoltageSourceConverterHVDCTrans/Control/Sending end and receiving end control/Receiving end control/Time mode/Measurements/Clarke ==
  abc : Inport
  0 : Fcn  Expr=u(1) + u(2) + u(3)
  K : Gain  Gain=[2 2 1]/3
  Mux : Mux  Inputs=3
  alpha : Fcn  Expr=(u(1) - u(3))*sqrt(3)/2
  beta : Fcn  Expr=-0.5*u(1) + u(2) -0.5*u(3)
  AlphaBeta0 : Outport
  wires:
  K/1 -> AlphaBeta0/1
  0/1 -> Mux/3
  alpha/1 -> Mux/1
  abc/1 -> 0/1, beta/1, alpha/1
  Mux/1 -> K/1
  beta/1 -> Mux/2

== system VoltageSourceConverterHVDCTrans/Control/Sending end and receiving end control/Receiving end control/Time mode/Measurements/Clarke1 ==
  abc : Inport
  0 : Fcn  Expr=u(1) + u(2) + u(3)
  K : Gain  Gain=[2 2 1]/3
  Mux : Mux  Inputs=3
  alpha : Fcn  Expr=(u(1) - u(3))*sqrt(3)/2
  beta : Fcn  Expr=-0.5*u(1) + u(2) -0.5*u(3)
  AlphaBeta0 : Outport
  wires:
  beta/1 -> Mux/2
  Mux/1 -> K/1
  abc/1 -> alpha/1, beta/1, 0/1
  alpha/1 -> Mux/1
  0/1 -> Mux/3
  K/1 -> AlphaBeta0/1

== system VoltageSourceConverterHVDCTrans/Control/Sending end and receiving end control/Receiving end control/Time mode/Measurements/PQ Calculation ==
  Vd : Inport
  Id : Inport  Port=2
  Iq : Inport  Port=3
  Gain : Gain  Gain=-1
  Product : Product
  Product4 : Product
  P : Outport
  Q : Outport  Port=2
  wires:
  Gain/1 -> Q/1
  Product4/1 -> Gain/1
  Iq/1 -> Product4/2
  Id/1 -> Product/2
  Product/1 -> P/1
  Vd/1 -> Product/1, Product4/1

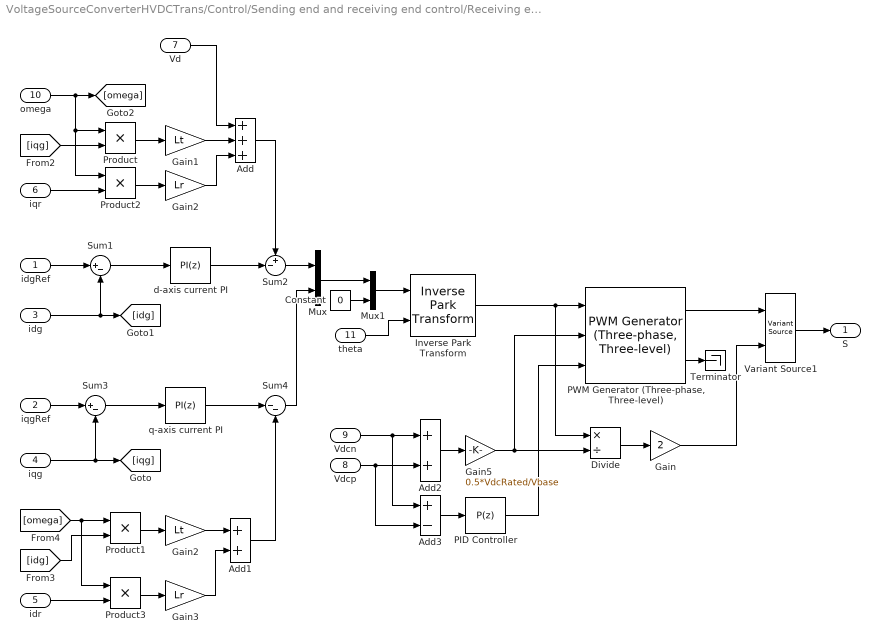
== system VoltageSourceConverterHVDCTrans/Control/Sending end and receiving end control/Receiving end control/Time mode/Receiving-end Control/Current control ==
  idgRef : Inport
  iqgRef : Inport  Port=2
  idg : Inport  Port=3
  iqg : Inport  Port=4
  idr : Inport  Port=5
  iqr : Inport  Port=6
  Vd : Inport  Port=7
  Vdcp : Inport  Port=8
  Vdcn : Inport  Port=9
  omega : Inport  Port=10
  theta : Inport  Port=11
  Add : Sum  Inputs=+++
  Add1 : Sum
  Add2 : Sum
  Add3 : Sum  Inputs=+-
  Constant : Constant  Value=0  SampleTime=Tsc
  Divide : Product  Inputs=*/
  Gain : Gain  Gain=2
  Gain1 : Gain  Gain=Lt
  Gain2 : Gain  Gain=Lr
  "Gain2 " : Gain  Gain=Lt
  Gain3 : Gain  Gain=Lr
  Gain5 : Gain  Gain=0.5*VdcRated/Vbase
  Inverse Park Transform : eeTransforms/Inverse Park Transform  AxisAlignment=Q-axis  PowerInvariant=off
  Mux : Mux  Inputs=2
  Mux1 : Mux  Inputs=2
  PID Controller : slpidlib/PID Controller  Controller=P  Form=Parallel  TimeDomain=Discrete-time  UseExternalTs=off  SampleTime=Tsc  IntegratorMethod=Forward Euler  FilterMethod=Forward Euler  ControllerParametersSource=internal  P=REnd_VdcB_P  I=1  UseKiTs=off  D=0  UseExternalDerivativeSource=off  N=100  UseFilter=on  TunerSelectOption=Transfer Function Based (PID Tuner App)  InitialConditionSource=internal  InitialConditionForIntegrator=0  InitialConditionForFilter=0  DifferentiatorICPrevScaledInput=0  ExternalReset=none  TrackingMode=off  Kt=1  LimitOutput=on  SatLimitsSource=internal  UpperSaturationLimit=1  LowerSaturationLimit=-1  LinearizeAsGain=on  AntiWindupMode=none  Kb=1  LimitIntegrator=off  UpperIntegratorSaturationLimit=inf  LowerIntegratorSaturationLimit=-inf  POutMin=[]  POutMax=[]  IOutMin=[]  IOutMax=[]  DOutMin=[]  DOutMax=[]  NOutMin=[]  NOutMax=[]  SumOutMin=[]  SumOutMax=[]  SaturationOutMin=[]  SaturationOutMax=[]  PParamMin=[]  PParamMax=[]  IParamMin=[]  IParamMax=[]  DParamMin=[]  DParamMax=[]  NParamMin=[]  NParamMax=[]  KbParamMin=[]  KbParamMax=[]  KtParamMin=[]  KtParamMax=[]  KbOutMin=[]  KbOutMax=[]  KtOutMin=[]  KtOutMax=[]  IntegratorOutMin=[]  IntegratorOutMax=[]  FilterOutMin=[]  FilterOutMax=[]  SumI1OutMin=[]  SumI1OutMax=[]  SumI2OutMin=[]  SumI2OutMax=[]  SumI3OutMin=[]  SumI3OutMax=[]  SumI4OutMin=[]  SumI4OutMax=[]  SumDOutMin=[]  SumDOutMax=[]  DifferentiatorOutMin=[]  DifferentiatorOutMax=[]  FilterDiffOutCoefMin=[]  FilterDiffOutCoefMax=[]  ReciprocalOutMin=[]  ReciprocalOutMax=[]  SumDenOutMin=[]  SumDenOutMax=[]  SumNumOutMin=[]  SumNumOutMax=[]  DivideOutMin=[]  DivideOutMax=[]  UdiffTsProdOutMin=[]  UdiffTsProdOutMax=[]  NTsProdOutMin=[]  NTsProdOutMax=[]  UintegralTsProdOutMin=[]  UintegralTsProdOutMax=[]  UngainTsProdOutMin=[]  UngainTsProdOutMax=[]  ClampingZeroOutDataTypeStr=Inherit: Inherit via back propagation  ClampingZeroOutMin=[]  ClampingZeroOutMax=[]  FilterDenConstantOutDataTypeStr=Inherit: Inherit via back propagation  FilterDenConstantOutMin=[]  FilterDenConstantOutMax=[]  PCopyOutDataTypeStr=Inherit: Inherit via back propagation  PCopyOutMin=[]  PCopyOutMax=[]  NCopyOutDataTypeStr=Inherit: Inherit via back propagation  NCopyOutMin=[]  NCopyOutMax=[]  IntegratorContinuousStateAttributes=''  IntegratorStateMustResolveToSignalObject=off  IntegratorRTWStateStorageClass=Auto  FilterContinuousStateAttributes=''  FilterStateMustResolveToSignalObject=off  FilterRTWStateStorageClass=Auto  ParallelPVariant=InternalParameters  IdealPVariant=Disabled  IVariant=Disabled  DVariant=Disabled  IntegratorVariant=Disabled  SatVariant=Enabled  AWVariant=Disabled  PCopyVariant=Disabled  TRVariant=Disabled  FdbkBlocksVariant=Forward  IdealPFdbkVariant=Disabled  SatFdbkVariant=Disabled  DerivativeFilterVariant=Disabled  NVariant=Disabled  NCopyVariant=Disabled_SignalSpec  FilterICVariant=Disabled  IntegratorICVariant=Disabled  ExternalResetVariant=Disabled  TRSumVariant=Passthrough  SumFdbkVariant=Disabled  SumVariant=Passthrough_P  TsampFilterVariant=InternalTs  TsampNgainVariant=Passthrough  TsampIntegralVariant=Disabled_SignalSpec  ExternalSaturationOutDataTypeStr=Inherit: Same as second input  DerivativeSourceVariant=Disabled  PreIntVariant=InternalPreInt
  "PWM Generator (Three-phase, Three-level)" : eePwmGeneratorThreeLevel/PWM Generator (Three-phase, Three-level)  CPWMMode=SPWM: sinusoidal PWM  fsw=fsw  Ts=Ts
      settings: SamplingMode=Natural
      settings: LibrarySourceBlock=|
      | ee_sl_lib/Pulse Width
      | Modulation/PWM Generator
      | (Three-phase, Three-level)
  Product{,1..3} (4 alike) : Product  Inputs=**
  Sum1 : Sum  Inputs=|+-
  Sum2 : Sum  Inputs=+-|
  Sum3 : Sum  Inputs=|+-
  Sum4 : Sum  Inputs=|--
  Terminator : Terminator
  Variant Source1 : VariantSource  ShowConditionOnBlock=on  VariantControls={SwitchingVSC, AverageValueVSC}
  d-axis current PI : slpidlib/PID Controller  Controller=PI  Form=Parallel  TimeDomain=Discrete-time  UseExternalTs=off  SampleTime=Tsc  IntegratorMethod=Forward Euler  FilterMethod=Forward Euler  ControllerParametersSource=internal  P=REnd_Id_PI(1)  I=REnd_Id_PI(2)  UseKiTs=off  D=0  UseExternalDerivativeSource=off  N=100  UseFilter=on  TunerSelectOption=Transfer Function Based (PID Tuner App)  InitialConditionSource=internal  InitialConditionForIntegrator=Id_PIr0  InitialConditionForFilter=0  DifferentiatorICPrevScaledInput=0  ExternalReset=none  TrackingMode=off  Kt=1  LimitOutput=on  SatLimitsSource=internal  UpperSaturationLimit=(Rt+Rr)*40  LowerSaturationLimit=-(Rt+Rr)*40  LinearizeAsGain=on  AntiWindupMode=back-calculation  Kb=1000  LimitIntegrator=off  UpperIntegratorSaturationLimit=0.18  LowerIntegratorSaturationLimit=-0.18  POutMin=[]  POutMax=[]  IOutMin=[]  IOutMax=[]  DOutMin=[]  DOutMax=[]  NOutMin=[]  NOutMax=[]  SumOutMin=[]  SumOutMax=[]  SaturationOutMin=[]  SaturationOutMax=[]  PParamMin=[]  PParamMax=[]  IParamMin=[]  IParamMax=[]  DParamMin=[]  DParamMax=[]  NParamMin=[]  NParamMax=[]  KbParamMin=[]  KbParamMax=[]  KtParamMin=[]  KtParamMax=[]  KbOutMin=[]  KbOutMax=[]  KtOutMin=[]  KtOutMax=[]  IntegratorOutMin=[]  IntegratorOutMax=[]  FilterOutMin=[]  FilterOutMax=[]  SumI1OutMin=[]  SumI1OutMax=[]  SumI2OutMin=[]  SumI2OutMax=[]  SumI3OutMin=[]  SumI3OutMax=[]  SumI4OutMin=[]  SumI4OutMax=[]  SumDOutMin=[]  SumDOutMax=[]  DifferentiatorOutMin=[]  DifferentiatorOutMax=[]  FilterDiffOutCoefMin=[]  FilterDiffOutCoefMax=[]  ReciprocalOutMin=[]  ReciprocalOutMax=[]  SumDenOutMin=[]  SumDenOutMax=[]  SumNumOutMin=[]  SumNumOutMax=[]  DivideOutMin=[]  DivideOutMax=[]  UdiffTsProdOutMin=[]  UdiffTsProdOutMax=[]  NTsProdOutMin=[]  NTsProdOutMax=[]  UintegralTsProdOutMin=[]  UintegralTsProdOutMax=[]  UngainTsProdOutMin=[]  UngainTsProdOutMax=[]  ClampingZeroOutDataTypeStr=Inherit: Inherit via back propagation  ClampingZeroOutMin=[]  ClampingZeroOutMax=[]  FilterDenConstantOutDataTypeStr=Inherit: Inherit via back propagation  FilterDenConstantOutMin=[]  FilterDenConstantOutMax=[]  PCopyOutDataTypeStr=Inherit: Inherit via back propagation  PCopyOutMin=[]  PCopyOutMax=[]  NCopyOutDataTypeStr=Inherit: Inherit via back propagation  NCopyOutMin=[]  NCopyOutMax=[]  IntegratorContinuousStateAttributes=''  IntegratorStateMustResolveToSignalObject=off  IntegratorRTWStateStorageClass=Auto  FilterContinuousStateAttributes=''  FilterStateMustResolveToSignalObject=off  FilterRTWStateStorageClass=Auto  ParallelPVariant=InternalParameters  IdealPVariant=Disabled  IVariant=InternalParameters  DVariant=Disabled  IntegratorVariant=Discrete  SatVariant=Enabled  AWVariant=BackCalculation  PCopyVariant=Disabled  TRVariant=Disabled  FdbkBlocksVariant=Forward  IdealPFdbkVariant=Disabled  SatFdbkVariant=Disabled  DerivativeFilterVariant=Disabled  NVariant=Disabled  NCopyVariant=Disabled_SignalSpec  FilterICVariant=Disabled  IntegratorICVariant=InternalICs  ExternalResetVariant=Disabled  TRSumVariant=Passthrough  SumFdbkVariant=Disabled  SumVariant=Sum_PI  TsampFilterVariant=InternalTs  TsampNgainVariant=Passthrough  TsampIntegralVariant=Disabled_SignalSpec  ExternalSaturationOutDataTypeStr=Inherit: Same as second input  DerivativeSourceVariant=Disabled  PreIntVariant=InternalPreInt
  q-axis current PI : slpidlib/PID Controller  Controller=PI  Form=Parallel  TimeDomain=Discrete-time  UseExternalTs=off  SampleTime=Tsc  IntegratorMethod=Forward Euler  FilterMethod=Forward Euler  ControllerParametersSource=internal  P=REnd_Iq_PI(1)  I=REnd_Iq_PI(2)  UseKiTs=off  D=0  UseExternalDerivativeSource=off  N=100  UseFilter=on  TunerSelectOption=Transfer Function Based (PID Tuner App)  InitialConditionSource=internal  InitialConditionForIntegrator=Iq_PIr0  InitialConditionForFilter=0  DifferentiatorICPrevScaledInput=0  ExternalReset=none  TrackingMode=off  Kt=1  LimitOutput=on  SatLimitsSource=internal  UpperSaturationLimit=(Rt+Rr)*40  LowerSaturationLimit=-(Rt+Rr)*40  LinearizeAsGain=on  AntiWindupMode=back-calculation  Kb=1000  LimitIntegrator=off  UpperIntegratorSaturationLimit=0.18  LowerIntegratorSaturationLimit=-0.18  POutMin=[]  POutMax=[]  IOutMin=[]  IOutMax=[]  DOutMin=[]  DOutMax=[]  NOutMin=[]  NOutMax=[]  SumOutMin=[]  SumOutMax=[]  SaturationOutMin=[]  SaturationOutMax=[]  PParamMin=[]  PParamMax=[]  IParamMin=[]  IParamMax=[]  DParamMin=[]  DParamMax=[]  NParamMin=[]  NParamMax=[]  KbParamMin=[]  KbParamMax=[]  KtParamMin=[]  KtParamMax=[]  KbOutMin=[]  KbOutMax=[]  KtOutMin=[]  KtOutMax=[]  IntegratorOutMin=[]  IntegratorOutMax=[]  FilterOutMin=[]  FilterOutMax=[]  SumI1OutMin=[]  SumI1OutMax=[]  SumI2OutMin=[]  SumI2OutMax=[]  SumI3OutMin=[]  SumI3OutMax=[]  SumI4OutMin=[]  SumI4OutMax=[]  SumDOutMin=[]  SumDOutMax=[]  DifferentiatorOutMin=[]  DifferentiatorOutMax=[]  FilterDiffOutCoefMin=[]  FilterDiffOutCoefMax=[]  ReciprocalOutMin=[]  ReciprocalOutMax=[]  SumDenOutMin=[]  SumDenOutMax=[]  SumNumOutMin=[]  SumNumOutMax=[]  DivideOutMin=[]  DivideOutMax=[]  UdiffTsProdOutMin=[]  UdiffTsProdOutMax=[]  NTsProdOutMin=[]  NTsProdOutMax=[]  UintegralTsProdOutMin=[]  UintegralTsProdOutMax=[]  UngainTsProdOutMin=[]  UngainTsProdOutMax=[]  ClampingZeroOutDataTypeStr=Inherit: Inherit via back propagation  ClampingZeroOutMin=[]  ClampingZeroOutMax=[]  FilterDenConstantOutDataTypeStr=Inherit: Inherit via back propagation  FilterDenConstantOutMin=[]  FilterDenConstantOutMax=[]  PCopyOutDataTypeStr=Inherit: Inherit via back propagation  PCopyOutMin=[]  PCopyOutMax=[]  NCopyOutDataTypeStr=Inherit: Inherit via back propagation  NCopyOutMin=[]  NCopyOutMax=[]  IntegratorContinuousStateAttributes=''  IntegratorStateMustResolveToSignalObject=off  IntegratorRTWStateStorageClass=Auto  FilterContinuousStateAttributes=''  FilterStateMustResolveToSignalObject=off  FilterRTWStateStorageClass=Auto  ParallelPVariant=InternalParameters  IdealPVariant=Disabled  IVariant=InternalParameters  DVariant=Disabled  IntegratorVariant=Discrete  SatVariant=Enabled  AWVariant=BackCalculation  PCopyVariant=Disabled  TRVariant=Disabled  FdbkBlocksVariant=Forward  IdealPFdbkVariant=Disabled  SatFdbkVariant=Disabled  DerivativeFilterVariant=Disabled  NVariant=Disabled  NCopyVariant=Disabled_SignalSpec  FilterICVariant=Disabled  IntegratorICVariant=InternalICs  ExternalResetVariant=Disabled  TRSumVariant=Passthrough  SumFdbkVariant=Disabled  SumVariant=Sum_PI  TsampFilterVariant=InternalTs  TsampNgainVariant=Passthrough  TsampIntegralVariant=Disabled_SignalSpec  ExternalSaturationOutDataTypeStr=Inherit: Same as second input  DerivativeSourceVariant=Disabled  PreIntVariant=InternalPreInt
  S : Outport
  wires:
  Gain/1 -> Variant Source1/2
  "PWM Generator (Three-phase, Three-level)"/2 -> Terminator/1
  Mux/1 -> Mux1/1
  iqgRef/1 -> Sum3/1
  Vd/1 -> Add/1
  idgRef/1 -> Sum1/1
  [idg] -> Product1/2
  Constant/1 -> Mux1/2
  Inverse Park Transform/1 -> Divide/1, "PWM Generator (Three-phase, Three-level)"/1
  Mux1/1 -> Inverse Park Transform/1
  [iqg] -> Product/2
  omega/1 -> Product2/1, Product/1, [omega]
  [omega] -> Product3/1, Product1/1
  Product/1 -> Gain1/1
  Sum4/1 -> Mux/2
  Product1/1 -> "Gain2 "/1
  Add/1 -> Sum2/1
  idg/1 -> Sum1/2, [idg]
  theta/1 -> Inverse Park Transform/2
  Gain1/1 -> Add/2
  Sum2/1 -> Mux/1
  iqr/1 -> Product2/2
  Product2/1 -> Gain2/1
  Gain2/1 -> Add/3
  idr/1 -> Product3/2
  Product3/1 -> Gain3/1
  "Gain2 "/1 -> Add1/1
  Gain3/1 -> Add1/2
  Add1/1 -> Sum4/2
  Variant Source1/1 -> S/1
  Divide/1 -> Gain/1
  "PWM Generator (Three-phase, Three-level)"/1 -> Variant Source1/1
  iqg/1 -> [iqg], Sum3/2
  d-axis current PI/1 -> Sum2/2
  Sum1/1 -> d-axis current PI/1
  q-axis current PI/1 -> Sum4/1
  Sum3/1 -> q-axis current PI/1
  Add2/1 -> Gain5/1
  Gain5/1 -> "PWM Generator (Three-phase, Three-level)"/2, Divide/2
  Vdcp/1 -> Add2/2, Add3/2
  Vdcn/1 -> Add2/1, Add3/1
  PID Controller/1 -> "PWM Generator (Three-phase, Three-level)"/3
  Add3/1 -> PID Controller/1
